simulink model "Solar_3S_Battery_System"  (R2021a)
settings: Solver=VariableStepAuto  StartTime=0.0  StopTime=10  RelTol=1e-3
libraries: nesl_utility x4, fl_lib x2, ee_lib x2, eeStairGenerator x1
settings Model: Creator=Invention  LastModifiedBy=Invention

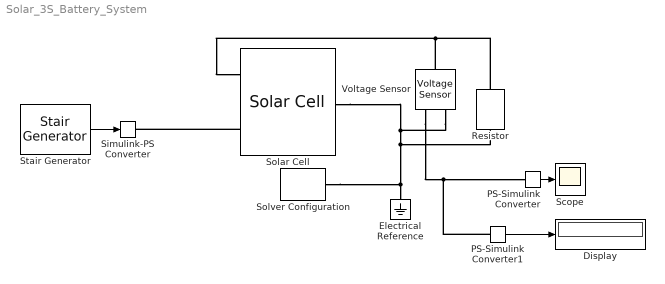
== system Solar_3S_Battery_System ==
  Display : Display
  Electrical Reference : fl_lib/Electrical/Electrical Elements/Electrical Reference
  PS-Simulink Converter : nesl_utility/PS-Simulink Converter  PhysicalDomain=network_engine_domain  SubClassName=ps_output  LeftPortType=input  RightPortType=output  PseudoPeriodic=off  Frequencies=[]  Unit=inherit  AffineConversion=off
      settings: SourceProductBaseCode=PW,SS
  PS-Simulink Converter1 : nesl_utility/PS-Simulink Converter  PhysicalDomain=network_engine_domain  SubClassName=ps_output  LeftPortType=input  RightPortType=output  PseudoPeriodic=off  Frequencies=[]  Unit=inherit  AffineConversion=off
      settings: SourceProductBaseCode=PW,SS
  Resistor : ee_lib/Passive/Resistor  R=10 Ohm  R_tol=5  enable_R_tol=0  tol_distribution=1  nSigma=4  enable_operating_limits=0  operating_limit_action=2  max_working_voltage=100 V  power_rating=1 W  enable_faults=0  fault_action=1  R_faulted=inf Ohm  enable_temporal_fault=0  t_fault=1 s  enable_behavioral_fault=0  max_permissible_current=1 A  t_fail_on_current=1 s  noise_mode=0  sample_time=1e-3 s  repeatability=1  auto_seed=4111000739  user_seed=0  Tdevice=25 degC  alpha=3.93e-3 1/K  Tmeas=25 degC  thermal_mass=100 J/K  power_derating_T1=70 degC  power_derating_T2=155 degC  operating_temperature_range_vec=[-50, 150] degC  temperature_specify=off  temperature_priority=High  temperature=298.15 K  temperature_nominal_specify=off  temperature_nominal_unit=K  temperature_nominal_value=1
  Scope : Scope
  Simulink-PS Converter : nesl_utility/Simulink-PS Converter  PhysicalDomain=network_engine_domain  SubClassName=ps_input  LeftPortType=input  RightPortType=output  PseudoPeriodic=off  Frequencies=[]  NoiseDistribution=none  NoiseParameters=[]  Unit=1  AffineConversion=off  FilteringAndDerivatives=provide  SimscapeFilterOrder=1  InputFilterTimeConstant=0.001  UdotUserProvided=0
      settings: SourceProductBaseCode=PW,SS
  Solar Cell : ee_lib/Sources/Solar Cell  prm=1  Isc=7.34 A  Voc=0.6 V  Is=1e-6 A  Is2=0 A  Iph=7.34 A  Ir0=1000 W/m^2  ec=1.5  N2=2  Rs=0 Ohm  Rp=inf Ohm  N_series=33  TIPH1=0 1/K  EG=1.11 eV  TXIS1=3  TXIS2=3  TRS1=0  TRP1=0  Tmeas=25 degC  TFIXED=25 degC  thermal_mass=100 J/K  initial_temperature=25 degC
      settings: SourceProductBaseCode=PS
  Solver Configuration : nesl_utility/Solver Configuration  PhysicalDomain=network_engine_domain  SubClassName=solver  LeftPortType=input  RightPortType=generic  Tones=[]  Harmonics=[]  SimulateNoise=off  Profile=off  UseLocalSampling=off  EnableSwitchedLinearOptims=on  FrequencyDomain=off  UseCCode=off  RelTol=0.001  AbsTol=1e-06  MinStep=1e-09  ToWorkspace=off  RevertToSquareIcSolve=off  NumHomotopyIterations=100  PhasorMode=off  PhasorModeNumHarmonics=1  DoDC=off  ResidualTolerance=1e-09  UseLocalSolver=off  LocalSolverChoice=NE_BACKWARD_EULER_ADVANCER  LocalSolverSampleTime=0.001  DoFixedCost=off  MaxNonlinIter=3  MaxModeIter=2  ComputeImpulses=off  ImpulseIterations=2  LinearAlgebra=auto  EquationFormulation=NE_TIME_EF  DelaysMemoryBudget=1024  AutomaticFiltering=on  FilteringTimeConstant=0.001  PartitionStorageMethod=AS_NEEDED  PartitionMemoryBudget=1024  PartitionMethod=ROBUST
      settings: SourceProductBaseCode=PW,SS
  Stair Generator : eeStairGenerator/Stair Generator  LabelModeActiveChoice=Discrete  TimeInput=[0 0.2 0.4 0.6 0.8 1 1.5]  AmplitudeInput=[1000 1000 800 500 200 0 0]  SampleTime=0.01  RepeatPattern=off  OutDataTypeStr=double
      settings: SourceProductBaseCode=PS
  Voltage Sensor : fl_lib/Electrical/Electrical Sensors/Voltage Sensor
  wires:
  PS-Simulink Converter/1 -> Scope/1
  PS-Simulink Converter1/1 -> Display/1
  Stair Generator/1 -> Simulink-PS Converter/1
  connections:
  Solar Cell/RConn1 -- Voltage Sensor/RConn2 -- Resistor/RConn1 -- Solver Configuration/RConn1 -- Electrical Reference/LConn1
  Solar Cell/LConn1 -- Simulink-PS Converter/RConn1
  Resistor/LConn1 -- Voltage Sensor/LConn1 -- Solar Cell/LConn2
  Voltage Sensor/RConn1 -- PS-Simulink Converter1/LConn1 -- PS-Simulink Converter/LConn1
